simulink model "MTE484Lab2"  (R2024b)
settings: Solver=VariableStepAuto  StartTime=0.0  StopTime=10.0  RelTol=1e-3
settings Model: Creator=sebastianassuncao  LastModifiedBy=Alex V

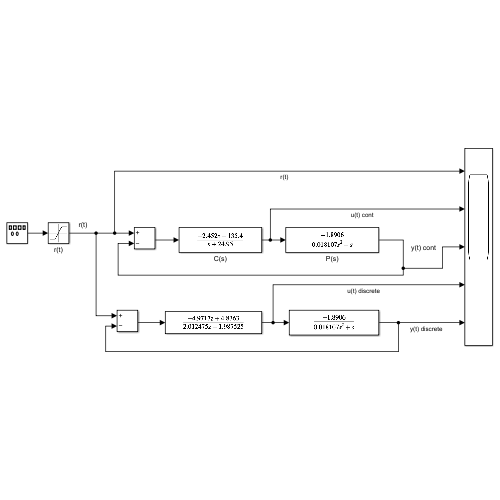
[thumbnail: Simulink's stored preview of the top-level diagram]
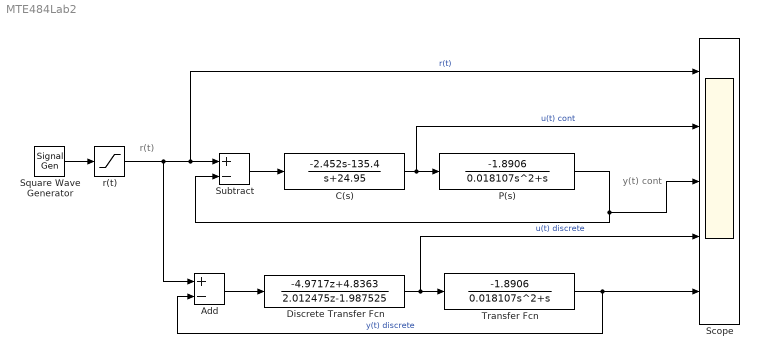
== system MTE484Lab2 ==
  note: y(t) cont
  note: r(t)
  Add : Sum  Inputs=+-
  C(s) : TransferFcn  Numerator=[-2.452 -135.4]  Denominator=[1 24.95]
  Discrete Transfer Fcn : DiscreteTransferFcn  Numerator=[-4.9717 4.8363]  Denominator=[2.012475 -1.987525]  SampleTime=0.0005
  P(s) : TransferFcn  Numerator=[-1.8906]  Denominator=[0.018107 1 0]
  Scope : Scope  NumInputPorts=5
  Square Wave Generator : SignalGenerator  WaveForm=square  Amplitude=2  Frequency=0.5
  Subtract : Sum  Inputs=+-
  Transfer Fcn : TransferFcn  Numerator=[-1.8906]  Denominator=[0.018107 1 0]
  r(t) : Saturate  UpperLimit=0.7  LowerLimit=-0.7
  wires:
  P(s)/1 -> Subtract/2, Scope/3
  r(t)/1 -> Add/1, Scope/1, Subtract/1  "r(t)"
  Square Wave Generator/1 -> r(t)/1
  Subtract/1 -> C(s)/1
  C(s)/1 -> Scope/2, P(s)/1  "u(t) cont"
  Add/1 -> Discrete Transfer Fcn/1
  Discrete Transfer Fcn/1 -> Scope/4, Transfer Fcn/1  "u(t) discrete"
  Transfer Fcn/1 -> Add/2, Scope/5  "y(t) discrete"
